simulink model "sanxiangqiaoshiquankongzhengliudianlu_R"  (R2025a)
settings: Solver=VariableStepAuto  StartTime=0.0  StopTime=0.2  RelTol=1e-3
libraries: spsThyristorLib x6, spsMultimeterLib x2, spsMeanLib x1, spsSeriesRLCBranchLib x1, spsThreePhaseVIMeasurementLib x1, spsThreePhaseSourceLib x1, sps_lib x1
settings Model: Creator=hdl  LastModifiedBy=hdl

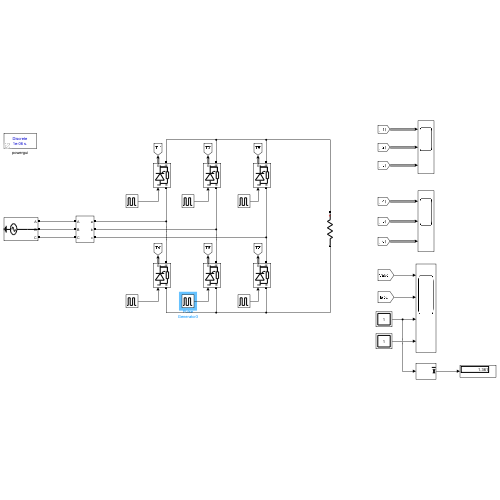
[thumbnail: Simulink's stored preview of the top-level diagram]
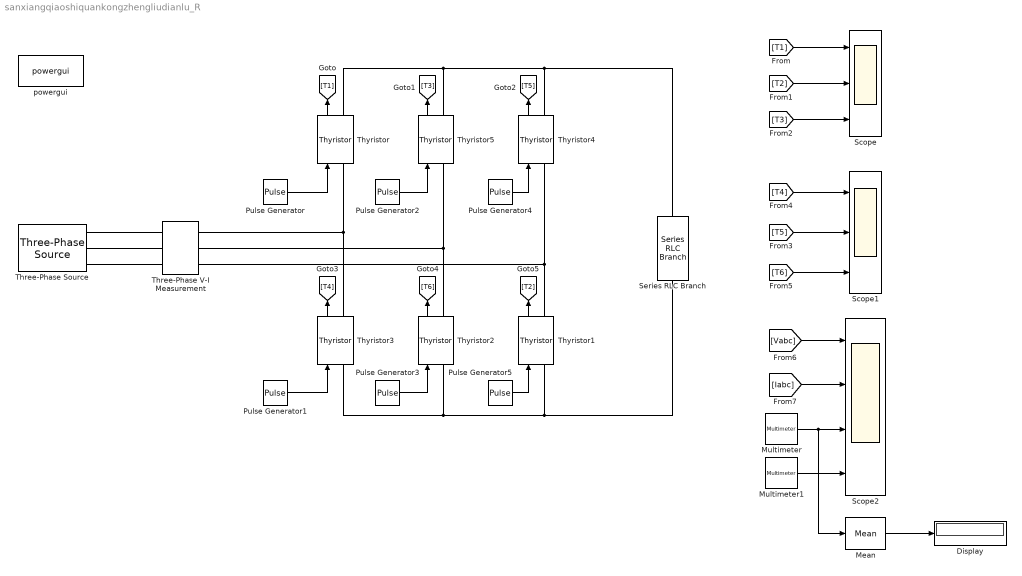
== system sanxiangqiaoshiquankongzhengliudianlu_R ==
  Display : Display
  Mean : spsMeanLib/Mean  Freq=60  Vinit=0  Ts=0
  Multimeter : spsMultimeterLib/Multimeter  L=2  sel=1  yselected={}  Gain=1  OutputType=Complex  PlotAtSimulationStop=off  PhasorSimulation=off
  Multimeter1 : spsMultimeterLib/Multimeter  L=2  sel=2  yselected={}  Gain=1  OutputType=Complex  PlotAtSimulationStop=off  PhasorSimulation=off
  Pulse Generator : DiscretePulseGenerator  PulseType=Time based  Period=0.02  PulseWidth=20  PhaseDelay=90/360*0.02
  Pulse Generator1 : DiscretePulseGenerator  PulseType=Time based  Period=0.02  PulseWidth=20  PhaseDelay=(180+90)/360*0.02
  Pulse Generator2 : DiscretePulseGenerator  PulseType=Time based  Period=0.02  PulseWidth=20  PhaseDelay=(120+90)/360*0.02
  Pulse Generator3 : DiscretePulseGenerator  PulseType=Time based  Period=0.02  PulseWidth=20  PhaseDelay=(120+180+90)/360*0.02
  Pulse Generator4 : DiscretePulseGenerator  PulseType=Time based  Period=0.02  PulseWidth=20  PhaseDelay=(240+90)/360*0.02
  Pulse Generator5 : DiscretePulseGenerator  PulseType=Time based  Period=0.02  PulseWidth=20  PhaseDelay=(240+180+90)/360*0.02
  Scope : Scope  NumInputPorts=3
      settings: ActiveDisplayYMinimum=-624.73727699367123  ActiveDisplayYMaximum=242.2949275595995
  Scope1 : Scope  NumInputPorts=3
  Scope2 : Scope  NumInputPorts=4
      settings: ActiveDisplayYMinimum=-403.89641198532354  ActiveDisplayYMaximum=429.48513791373608  DataLoggingVariableName=ScopeData2
  Series RLC Branch : spsSeriesRLCBranchLib/Series RLC Branch  LConnTagsString=__new0  RConnTagsString=__new0  BranchType=R  Resistance=10  Inductance=1e-3  SetiL0=off  InitialCurrent=0  Capacitance=1e-6  Setx0=off  InitialVoltage=0  Measurements=Branch voltage and current
  Three-Phase V-I Measurement : spsThreePhaseVIMeasurementLib/Three-Phase V-I Measurement  VoltageMeasurement=phase-to-ground  SetLabelV=on  LabelV=Vabc  Vpu=off  VpuLL=off  CurrentMeasurement=yes  SetLabelI=on  LabelI=Iabc  Ipu=off  Pbase=100e6  Vbase=500e3  OutputType=Complex  PhasorSimulation=off  PSBequivalent=0
  Three-Phase Source : spsThreePhaseSourceLib/Three-Phase Source  InternalConnection=Yg  VoltagePhases=off  Voltage=220*sqrt(3)  PhaseAngle=0  Voltage_phases=[25e3 25e3 25e3]/sqrt(3)  PhaseAngles_phases=[0 -120 +120]  Frequency=50  NonIdealSource=off  SpecifyImpedance=off  Resistance=0.8929  Inductance=16.58e-3  ShortCircuitLevel=100e6  BaseVoltage=25e3  XRratio=7  BusType=swing  Pref=10e3  Qref=0  Prefabc=[10e3, 10e3, 10e3]  Qrefabc=[0, 0, 0]  Qmin=-inf  Qmax=inf
  Thyristor{,1..5} (6 alike) : spsThyristorLib/Thyristor  Ron=0.001  Lon=0  Vf=0.8  IC=0  Rs=500  Cs=250e-9  Measurements=on
  powergui : sps_lib/powergui  Priority=1  SimulationMode=Discrete  SampleTime=1e-6  frequency=60  Iterations=50  frequencyindice=50  Pbase=100e6  ErrMax=1e-4  UnitsV=kV  UnitsW=MW  buscounter=0  FunctionMessages=off  echomessages=off  EnableUseOfTLC=off  CurrentSourceSwitches=off  DisableSnubberDevices=off  DisableRonSwitches=off  DisableVfSwitches=off  DisplayEquations=off  AutomaticDiscreteSolvers=off  SolverType=Tustin/Backward Euler (TBE)  Interpol=off  ExternalGateDelay=off  methode=off  Ts=100  x0status=blocks  SPID=on  SwTol=0  HookPort=off  NonlinearTolerance=1e-4  nMaxIteration=100  ContinueOnMaxIteration=off  RestoreLinks=warning  ResistiveCurrentMeasurement=off  Frange=[0:2:500]  Ylog=off  Xlog=on  ShowGrid=off  save=off  variable=ZData  structure=0  ZoomFFT=off  StartTime=0.0  cycles=1  DisplayStyle=1  fundamental=60  FreqAxis=off  MaxFrequency=1000  frequencyindicesteady=1  RmsSteady=1  display=off
  wires:
  Pulse Generator/1 -> Thyristor/1
  Pulse Generator1/1 -> Thyristor3/1
  Pulse Generator2/1 -> Thyristor5/1
  Pulse Generator4/1 -> Thyristor4/1
  Pulse Generator5/1 -> Thyristor1/1
  Thyristor/1 -> [T1]
  Thyristor5/1 -> [T3]
  Thyristor4/1 -> [T5]
  Thyristor3/1 -> [T4]
  Thyristor2/1 -> [T6]
  Thyristor1/1 -> [T2]
  [T1] -> Scope/1
  [T2] -> Scope/2
  [T3] -> Scope/3
  [T4] -> Scope1/1
  [T5] -> Scope1/2
  [T6] -> Scope1/3
  Mean/1 -> Display/1
  Multimeter1/1 -> Scope2/4
  Multimeter/1 -> Mean/1, Scope2/3
  [Iabc] -> Scope2/2
  [Vabc] -> Scope2/1
  Pulse Generator3/1 -> Thyristor2/1
  connections:
  Three-Phase V-I Measurement/LConn3 -- Three-Phase Source/RConn3
  Three-Phase V-I Measurement/LConn2 -- Three-Phase Source/RConn2
  Three-Phase V-I Measurement/LConn1 -- Three-Phase Source/RConn1
  Thyristor/LConn1 -- Three-Phase V-I Measurement/RConn1 -- Thyristor3/RConn1
  Thyristor5/LConn1 -- Three-Phase V-I Measurement/RConn2 -- Thyristor2/RConn1
  Thyristor4/LConn1 -- Three-Phase V-I Measurement/RConn3 -- Thyristor1/RConn1
  Thyristor/RConn1 -- Thyristor5/RConn1 -- Series RLC Branch/LConn1 -- Thyristor4/RConn1
  Thyristor3/LConn1 -- Thyristor2/LConn1 -- Series RLC Branch/RConn1 -- Thyristor1/LConn1
